simulink model "induction_machine_skalarne_R2025a"  (R2025a)
settings: Solver=FixedStepAuto  StopTime=10  FixedStep=Ts
PreLoadFcn:
  | Ts = 250e-6;
InitFcn:
  | Ts = 250e-6;
libraries: autolibim x1
settings Model: Creator=Kajo  LastModifiedBy=patrikmitro
settings SFSimCC: SimGPUStackLimitPerThread=51200  SimGPUMallocThreshold=200
settings RTWCC: GPUStackLimitPerThread=51200  GPUMallocThreshold=200

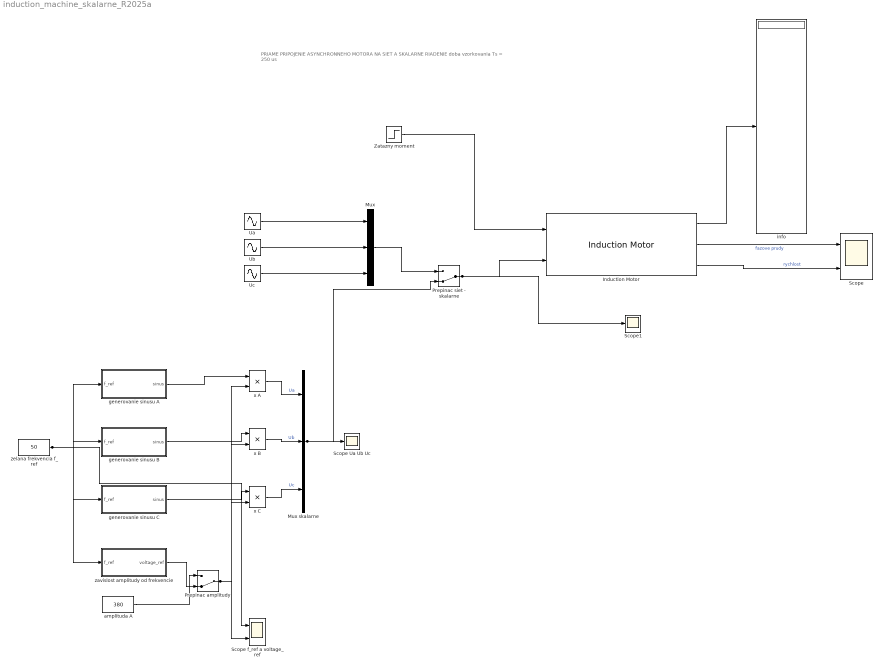
== system induction_machine_skalarne_R2025a ==
  note: PRIAME PRIPOJENIE ASYNCHRONNEHO MOTORA NA SIET A SKALARNE RIADENIE
      | doba vzorkovania Ts = 250 us
  Induction Motor : autolibim/Induction Motor  sim_type=Continuous  Ts=0.001  port_config=Torque  P=1  Zs=[4.36 0.013]  Zr="[2.16  0.013]"  Lm=0.46  mechanical=[0.0017 0.001 0]  theta_init=0  omega_init=0  RefBlkName='autolibim/Induction Motor'  aMode=5
      settings: LibrarySourceBlock=mcblib/Control/Induction Machine/Electrical Systems/Motors/Induction Motor
  Mux : Mux  Inputs=3
  Mux skalarne : Mux  Inputs=3
  Prepinac amplitudy : ManualSwitch  CurrentSetting=0
  Prepinac siet - skalarne : ManualSwitch  CurrentSetting=0
  Scope : Scope  NumInputPorts=2
      settings: ActiveDisplayYMinimum=-46.747236547829374  ActiveDisplayYMaximum=50.780413986284138
  Scope Ua Ub Uc : Scope
  Scope f_ref a voltage_ref : Scope  NumInputPorts=2
  Scope1 : Scope
      settings: ActiveDisplayYMinimum=-475  ActiveDisplayYMaximum=475
  Ua : Sin  Amplitude=380  Frequency=2*pi*50  SampleTime=0
  Ub : Sin  Amplitude=380  Frequency=2*pi*50  Phase=-(2*pi)/3  SampleTime=0
  Uc : Sin  Amplitude=380  Frequency=2*pi*50  Phase=-(4*pi)/3  SampleTime=0
  Zatazny moment : Step  Time=2  After=4.98  SampleTime=0
  amplituda A : Constant  Value=380
  generovanie sinusu A : Subsystem
  generovanie sinusu B : Subsystem
  generovanie sinusu C : Subsystem
  info : Display
  x A : Product
  x B : Product
  x C : Product
  zavislost amplitudy od frekvencie : MATLAB Function  TreatAsAtomicUnit=on
  zelana frekvencia f_ref : Constant  Value=50
  wires:
  Ua/1 -> Mux/1
  Ub/1 -> Mux/2
  Uc/1 -> Mux/3
  Zatazny moment/1 -> Induction Motor/1
  Induction Motor/2 -> Scope/1  "fazove prudy"
  Induction Motor/3 -> Scope/2  "rychlost"
  Induction Motor/1 -> info/1
  zelana frekvencia f_ref/1 -> generovanie sinusu A/1(f_ref), generovanie sinusu B/1(f_ref), generovanie sinusu C/1(f_ref), zavislost amplitudy od frekvencie/1(f_ref), Scope f_ref a voltage_ref/1
  amplituda A/1 -> Prepinac amplitudy/1
  zavislost amplitudy od frekvencie/1(voltage_ref) -> Prepinac amplitudy/2
  Prepinac amplitudy/1 -> Scope f_ref a voltage_ref/2, x A/2, x B/2, x C/2
  generovanie sinusu A/1(sinus) -> x A/1
  x A/1 -> Mux skalarne/1  "Ua"
  generovanie sinusu B/1(sinus) -> x B/1
  x B/1 -> Mux skalarne/2  "Ub"
  generovanie sinusu C/1(sinus) -> x C/1
  x C/1 -> Mux skalarne/3  "Uc"
  Mux skalarne/1 -> Scope Ua Ub Uc/1, Prepinac siet - skalarne/2
  Mux/1 -> Prepinac siet - skalarne/1
  Prepinac siet - skalarne/1 -> Induction Motor/2, Scope1/1

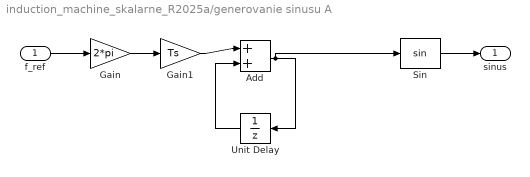
== system induction_machine_skalarne_R2025a/generovanie sinusu A ==
  f_ref : Inport
  Add : Sum
  Gain : Gain  Gain=2*pi
  Gain1 : Gain  Gain=Ts
  Sin : Trigonometry
  Unit Delay : UnitDelay  SampleTime=Ts
  sinus : Outport
  wires:
  f_ref/1 -> Gain/1
  Gain/1 -> Gain1/1
  Gain1/1 -> Add/1
  Add/1 -> Unit Delay/1, Sin/1
  Unit Delay/1 -> Add/2
  Sin/1 -> sinus/1

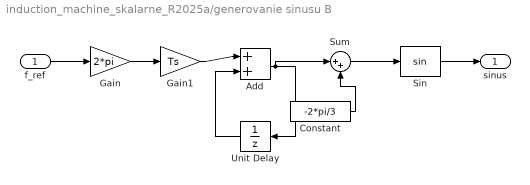
== system induction_machine_skalarne_R2025a/generovanie sinusu B ==
  f_ref : Inport
  Add : Sum
  Constant : Constant  Value=-2*pi/3
  Gain : Gain  Gain=2*pi
  Gain1 : Gain  Gain=Ts
  Sin : Trigonometry
  Sum : Sum  Inputs=|++
  Unit Delay : UnitDelay  SampleTime=Ts
  sinus : Outport
  wires:
  f_ref/1 -> Gain/1
  Gain/1 -> Gain1/1
  Gain1/1 -> Add/1
  Add/1 -> Unit Delay/1, Sum/1
  Unit Delay/1 -> Add/2
  Constant/1 -> Sum/2
  Sum/1 -> Sin/1
  Sin/1 -> sinus/1

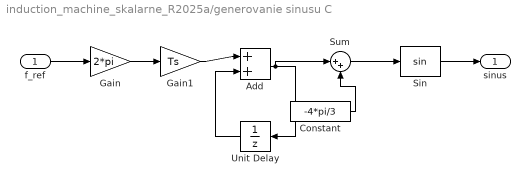
== system induction_machine_skalarne_R2025a/generovanie sinusu C ==
  f_ref : Inport
  Add : Sum
  Constant : Constant  Value=-4*pi/3
  Gain : Gain  Gain=2*pi
  Gain1 : Gain  Gain=Ts
  Sin : Trigonometry
  Sum : Sum  Inputs=|++
  Unit Delay : UnitDelay  SampleTime=Ts
  sinus : Outport
  wires:
  f_ref/1 -> Gain/1
  Gain/1 -> Gain1/1
  Gain1/1 -> Add/1
  Add/1 -> Unit Delay/1, Sum/1
  Unit Delay/1 -> Add/2
  Constant/1 -> Sum/2
  Sum/1 -> Sin/1
  Sin/1 -> sinus/1

== matlab function induction_machine_skalarne_R2025a/zavislost amplitudy od frekvencie ==
  data: f_ref input; voltage_ref output
function voltage_ref = fcn(f_ref)
% Zavislost amplitudy fazoveho napatia od frekvencie (obr. 1)
Un     = 380;          % amplituda napatia pri menovitej frekvencii [V]
fn     = 50;           % menovita frekvencia [Hz]
fb     = 3;            % hranica oblasti Uboost [Hz]
Uboost = Un/fn*fb;     % konstantne napatie pre 0..3 Hz (22,8 V)

if f_ref < 0
    voltage_ref = 0;               % f < 0 Hz: neplatna frekvencia
elseif f_ref <= fb
    voltage_ref = Uboost;          % 0..3 Hz: Uboost
elseif f_ref <= fn
    voltage_ref = Un/fn*f_ref;     % 3..50 Hz: U/f = konst.
else
    voltage_ref = Un;              % f > 50 Hz: napatie sa uz nezvysuje
end
end
